simulink model "ASM_Traffic_new"  (R2024a)
settings: Solver=ode1  StartTime=SIM.tstart.v  StopTime=SIM.tend.v  FixedStep=SIM.StepSize.v  RelTol=1e-3
PostLoadFcn:
  | if any(exist('dsrtsu_mdlpostloadfcn', 'file') ~= 0), dsrtsu_mdlpostloadfcn('Execute', bdroot); end
  | try, asm_mdl_postloadfcn(bdroot, 'UpdateModel', 3600); catch, disp(lasterr); end,
InitFcn:
  | , if any(exist('rtifpga_mdlclblib', 'file') ~= 0), rtifpga_mdlclblib('Init', bdroot); end,
  | , if any(exist('dsmpb_private', 'file') ~= 0), dsmpb_private('dsmpb_mdlclblib', 'Init', bdroot); end,
undefined symbols (not defined in the file): _to_, a0b2, ASM_BrakeHydraulics_DemoSystems, ASM_VehicleDynamics_DemoSystems, b98103fe8ad365046cd0, BrakeCircuit, CPT, Crankshaft, DiscIntNeverNeededParam, dsmsi, FinalDriveAssembly, MDL, ModeSignals, Pos_BrakePedal_Maneuver, rad, RefSignals, s_to_rpm, SIM, SoftECU, Suspension, Tire, Transmission
libraries: ASM_Traffic_lib x135, simulink x100, ASM_Utils_lib x77, ASM_VehicleDynamics_lib x70, ASM_Environment_lib x22, dsmpblib x20, dsmsilib x15, MDLD_Utils_lib x10, ASM_BrakeHydraulics_lib x3
(part 45 of 63)

== system ASM_Traffic_new/Drivetrain/Plant/UserInterface/DISP_Plant/ActiveTransmission/Trq_Out_Trm[Nm] ==
  In1 : Inport
  Out1 : Outport  VectorParamsAs1DForOutWhenUnconnected=off
  wires:
  In1/1 -> Out1/1

== system ASM_Traffic_new/Drivetrain/Plant/UserInterface/DISP_Plant/ActiveTransmission/i_Trm[] ==
  In1 : Inport
  Out1 : Outport  VectorParamsAs1DForOutWhenUnconnected=off
  wires:
  In1/1 -> Out1/1

== system ASM_Traffic_new/Drivetrain/Plant/UserInterface/DISP_Plant/ActiveTransmission/i_unsync_Trm[] ==
  In1 : Inport
  Out1 : Outport  VectorParamsAs1DForOutWhenUnconnected=off
  wires:
  In1/1 -> Out1/1

== system ASM_Traffic_new/Drivetrain/Plant/UserInterface/DISP_Plant/ActiveTransmission/omega_In_Trm[rad|s] ==
  In1 : Inport
  Out1 : Outport  VectorParamsAs1DForOutWhenUnconnected=off
  wires:
  In1/1 -> Out1/1

== system ASM_Traffic_new/Drivetrain/Plant/UserInterface/DISP_Plant/ActiveTransmission/omega_Out_Trm[rad|s] ==
  In1 : Inport
  Out1 : Outport  VectorParamsAs1DForOutWhenUnconnected=off
  wires:
  In1/1 -> Out1/1

== system ASM_Traffic_new/Drivetrain/Plant/UserInterface/DISP_Plant/AutomaticTransmission/Trq_Fric_Clutch[Nm] ==
  In1 : Inport
  Out1 : Outport  VectorParamsAs1DForOutWhenUnconnected=off
  wires:
  In1/1 -> Out1/1

== system ASM_Traffic_new/Drivetrain/Plant/UserInterface/DISP_Plant/AutomaticTransmission/Trq_Pump[Nm] ==
  In1 : Inport
  Out1 : Outport  VectorParamsAs1DForOutWhenUnconnected=off
  wires:
  In1/1 -> Out1/1

== system ASM_Traffic_new/Drivetrain/Plant/UserInterface/DISP_Plant/AutomaticTransmission/Trq_TorsionSpring_Clutch[Nm] ==
  In1 : Inport
  Out1 : Outport  VectorParamsAs1DForOutWhenUnconnected=off
  wires:
  In1/1 -> Out1/1

== system ASM_Traffic_new/Drivetrain/Plant/UserInterface/DISP_Plant/AutomaticTransmission/Trq_Turbine[Nm] ==
  In1 : Inport
  Out1 : Outport  VectorParamsAs1DForOutWhenUnconnected=off
  wires:
  In1/1 -> Out1/1

== system ASM_Traffic_new/Drivetrain/Plant/UserInterface/DISP_Plant/AutomaticTransmission/omega_Out_ClutchPlate[rad|s] ==
  In1 : Inport
  Out1 : Outport  VectorParamsAs1DForOutWhenUnconnected=off
  wires:
  In1/1 -> Out1/1

== system ASM_Traffic_new/Drivetrain/Plant/UserInterface/DISP_Plant/EngineSpeed/Trq_Starter[Nm] ==
  In1 : Inport
  Out1 : Outport  VectorParamsAs1DForOutWhenUnconnected=off
  wires:
  In1/1 -> Out1/1

== system ASM_Traffic_new/Drivetrain/Plant/UserInterface/DISP_Plant/EngineSpeed/n_Engine[rpm] ==
  In1 : Inport
  Out1 : Outport  VectorParamsAs1DForOutWhenUnconnected=off
  wires:
  In1/1 -> Out1/1

== system ASM_Traffic_new/Drivetrain/Plant/UserInterface/DISP_Plant/ManualTransmission/Trq_Fric_Clutch[Nm] ==
  In1 : Inport
  Out1 : Outport  VectorParamsAs1DForOutWhenUnconnected=off
  wires:
  In1/1 -> Out1/1

== system ASM_Traffic_new/Drivetrain/Plant/UserInterface/DISP_Plant/ManualTransmission/Trq_TorsionSpring_Clutch[Nm] ==
  In1 : Inport
  Out1 : Outport  VectorParamsAs1DForOutWhenUnconnected=off
  wires:
  In1/1 -> Out1/1

== system ASM_Traffic_new/Drivetrain/Plant/UserInterface/DISP_Plant/ManualTransmission/omega_Out_ClutchPlate[rad|s] ==
  In1 : Inport
  Out1 : Outport  VectorParamsAs1DForOutWhenUnconnected=off
  wires:
  In1/1 -> Out1/1

== system ASM_Traffic_new/Drivetrain/Plant/UserInterface/DISP_Plant/Shafts/Trq_CF_Shaft[Nm] ==
  In1 : Inport
  Out1 : Outport  VectorParamsAs1DForOutWhenUnconnected=off
  wires:
  In1/1 -> Out1/1

== system ASM_Traffic_new/Drivetrain/Plant/UserInterface/DISP_Plant/Shafts/Trq_CR_Shaft[Nm] ==
  In1 : Inport
  Out1 : Outport  VectorParamsAs1DForOutWhenUnconnected=off
  wires:
  In1/1 -> Out1/1

== system ASM_Traffic_new/Drivetrain/Plant/UserInterface/DISP_Plant/Shafts/Trq_FL_Shaft[Nm] ==
  In1 : Inport
  Out1 : Outport  VectorParamsAs1DForOutWhenUnconnected=off
  wires:
  In1/1 -> Out1/1

== system ASM_Traffic_new/Drivetrain/Plant/UserInterface/DISP_Plant/Shafts/Trq_FR_Shaft[Nm] ==
  In1 : Inport
  Out1 : Outport  VectorParamsAs1DForOutWhenUnconnected=off
  wires:
  In1/1 -> Out1/1

== system ASM_Traffic_new/Drivetrain/Plant/UserInterface/DISP_Plant/Shafts/Trq_RL_Shaft[Nm] ==
  In1 : Inport
  Out1 : Outport  VectorParamsAs1DForOutWhenUnconnected=off
  wires:
  In1/1 -> Out1/1

== system ASM_Traffic_new/Drivetrain/Plant/UserInterface/DISP_Plant/Shafts/Trq_RR_Shaft[Nm] ==
  In1 : Inport
  Out1 : Outport  VectorParamsAs1DForOutWhenUnconnected=off
  wires:
  In1/1 -> Out1/1

== system ASM_Traffic_new/Environment/GroundTruth/UserInterface/PAR_Plant/Ego_Vehicle/Indicator_State[] ==
  ASM_Vehicle_TurnLights[] : Inport
  ASM_OSI_Mapping : Subsystem
  Ext_Indicator_State[] : Constant  Value=0
  Multiport Switch : MultiPortSwitch  DataPortOrder=Zero-based contiguous  zeroidx=on  SaturateOnIntegerOverflow=off  InputSameDT=off
  Rounding Function : Rounding  Operator=round
  Saturation : Saturate  UpperLimit=2  LowerLimit=0
  Stim_Indicator_State[] : Constant  Value=0
  Sw_Indicator[0Stim|1Ext|2Mnv] : Constant  Value=2
  Indicator_State[] : Outport  VectorParamsAs1DForOutWhenUnconnected=off
  wires:
  ASM_OSI_Mapping/1(Indicator_State[]) -> Multiport Switch/4  "Mnv_Indicator_State[]"
  Stim_Indicator_State[]/1 -> Multiport Switch/2  "Stim_Indicator_State[]"
  Multiport Switch/1 -> Indicator_State[]/1  "Indicator_State[]"
  Saturation/1 -> Multiport Switch/1
  Rounding Function/1 -> Saturation/1
  Ext_Indicator_State[]/1 -> Multiport Switch/3  "Ext_Indicator_State[]"
  ASM_Vehicle_TurnLights[]/1 -> ASM_OSI_Mapping/1(ASM_Vehicle_TurnLights[])
  Sw_Indicator[0Stim|1Ext|2Mnv]/1 -> Rounding Function/1  "Sw_Indicator[0Stim|1Ext|2Mnv]"

== system ASM_Traffic_new/Environment/GroundTruth/UserInterface/PAR_Plant/Fellow_Vehicles/Demux_Fellow_Lightstates ==
  Fellow_Lightstates[] : Inport
  Add{,1..8} (9 alike) : Sum
  Constant : Constant
  Constant1 : Constant  Value=2
  Constant2 : Constant  Value=3
  Constant3 : Constant  Value=4
  Constant4 : Constant  Value=5
  Constant5 : Constant  Value=8
  Constant6 : Constant  Value=9
  Constant7 : Constant  Value=6
  Constant8 : Constant  Value=7
  Main_Idx_30Fellows : Constant  Value=[1,11,21,31,41,51,61,71,81,91,101,111,121,131,141,151,161,171,181,191,201,211,221,231,241,251,261,271,281,291]
  Selector_Brake_State[] : Selector  InputPortWidth=MDL.Traffic.MaxNumFellows.v*10  IndexOptions=Index vector (port)  Indices=[1 3]  OutputSizes=1
  Selector_Emergency_Veh_Illu[] : Selector  InputPortWidth=MDL.Traffic.MaxNumFellows.v*10  IndexOptions=Index vector (port)  Indices=[1 3]  OutputSizes=1
  Selector_Front_Fog_Light[] : Selector  InputPortWidth=MDL.Traffic.MaxNumFellows.v*10  IndexOptions=Index vector (port)  Indices=[1 3]  OutputSizes=1
  Selector_Head_Light[] : Selector  InputPortWidth=MDL.Traffic.MaxNumFellows.v*10  IndexOptions=Index vector (port)  Indices=[1 3]  OutputSizes=1
  Selector_High_Beam : Selector  InputPortWidth=MDL.Traffic.MaxNumFellows.v*10  IndexOptions=Index vector (port)  Indices=[1 3]  OutputSizes=1
  Selector_Indicator_State[] : Selector  InputPortWidth=MDL.Traffic.MaxNumFellows.v*10  IndexOptions=Index vector (port)  Indices=[1 3]  OutputSizes=1
  Selector_License_Plate_Illumination[] : Selector  InputPortWidth=MDL.Traffic.MaxNumFellows.v*10  IndexOptions=Index vector (port)  Indices=[1 3]  OutputSizes=1
  Selector_Rear_Fog_Light[] : Selector  InputPortWidth=MDL.Traffic.MaxNumFellows.v*10  IndexOptions=Index vector (port)  Indices=[1 3]  OutputSizes=1
  Selector_Reversing_Light[] : Selector  InputPortWidth=MDL.Traffic.MaxNumFellows.v*10  IndexOptions=Index vector (port)  Indices=[1 3]  OutputSizes=1
  Selector_Service_Veh_Illu[] : Selector  InputPortWidth=MDL.Traffic.MaxNumFellows.v*10  IndexOptions=Index vector (port)  Indices=[1 3]  OutputSizes=1
  High_Beam_Fellows[] : Outport  VectorParamsAs1DForOutWhenUnconnected=off
  Reversing_Light_Fellows[] : Outport  Port=2  VectorParamsAs1DForOutWhenUnconnected=off
  Front_Fog_Light_Fellows[] : Outport  Port=3  VectorParamsAs1DForOutWhenUnconnected=off
  Head_Light_Fellows[] : Outport  Port=4  VectorParamsAs1DForOutWhenUnconnected=off
  License_Plate_Illumination_Fellows[] : Outport  Port=5  VectorParamsAs1DForOutWhenUnconnected=off
  Rear_Fog_Light_Fellows[] : Outport  Port=6  VectorParamsAs1DForOutWhenUnconnected=off
  Emergency_Veh_Illu_Fellows[] : Outport  Port=7  VectorParamsAs1DForOutWhenUnconnected=off
  Service_Veh_Illu_Fellows[] : Outport  Port=8  VectorParamsAs1DForOutWhenUnconnected=off
  Indicator_State_Fellows[] : Outport  Port=9  VectorParamsAs1DForOutWhenUnconnected=off
  Brake_Fellows[] : Outport  Port=10  VectorParamsAs1DForOutWhenUnconnected=off
  wires:
  Fellow_Lightstates[]/1 -> Selector_Service_Veh_Illu[]/1, Selector_Brake_State[]/1, Selector_Indicator_State[]/1, Selector_Emergency_Veh_Illu[]/1, Selector_Rear_Fog_Light[]/1, Selector_License_Plate_Illumination[]/1, Selector_Head_Light[]/1, Selector_Front_Fog_Light[]/1, Selector_Reversing_Light[]/1, Selector_High_Beam/1
  Main_Idx_30Fellows/1 -> Add7/1, Add8/1, Add6/1, Add5/1, Add4/1, Add3/1, Add2/1, Add1/1, Add/1, Selector_High_Beam/2
  Selector_High_Beam/1 -> High_Beam_Fellows[]/1
  Add/1 -> Selector_Reversing_Light[]/2
  Constant/1 -> Add/2
  Selector_Reversing_Light[]/1 -> Reversing_Light_Fellows[]/1
  Selector_Front_Fog_Light[]/1 -> Front_Fog_Light_Fellows[]/1
  Add1/1 -> Selector_Front_Fog_Light[]/2
  Constant1/1 -> Add1/2
  Selector_Head_Light[]/1 -> Head_Light_Fellows[]/1
  Add2/1 -> Selector_Head_Light[]/2
  Constant2/1 -> Add2/2
  Selector_License_Plate_Illumination[]/1 -> License_Plate_Illumination_Fellows[]/1
  Add3/1 -> Selector_License_Plate_Illumination[]/2
  Constant3/1 -> Add3/2
  Selector_Rear_Fog_Light[]/1 -> Rear_Fog_Light_Fellows[]/1
  Add4/1 -> Selector_Rear_Fog_Light[]/2
  Constant4/1 -> Add4/2
  Selector_Indicator_State[]/1 -> Indicator_State_Fellows[]/1
  Add5/1 -> Selector_Indicator_State[]/2
  Constant5/1 -> Add5/2
  Selector_Brake_State[]/1 -> Brake_Fellows[]/1
  Add6/1 -> Selector_Brake_State[]/2
  Constant6/1 -> Add6/2
  Add7/1 -> Selector_Emergency_Veh_Illu[]/2
  Constant7/1 -> Add7/2
  Add8/1 -> Selector_Service_Veh_Illu[]/2
  Constant8/1 -> Add8/2
  Selector_Emergency_Veh_Illu[]/1 -> Emergency_Veh_Illu_Fellows[]/1
  Selector_Service_Veh_Illu[]/1 -> Service_Veh_Illu_Fellows[]/1

== system ASM_Traffic_new/Environment/GroundTruth/UserInterface/PAR_Plant/Fellow_Vehicles/Lightstates_Fellow1 ==
  Fellow_Indicator_State[] : Inport
  Brake[] : Constant  Tag=AD:ASM_Sw_SpeedLimit_Source[1Manual|2RoadScenery]  Value=2
  Emergency_Vehicle_Illumination[] : Constant  Tag=AD:ASM_Sw_SpeedLimit_Source[1Manual|2RoadScenery]  Value=2
  Front_Fog_Light[] : Constant  Tag=AD:ASM_Sw_SpeedLimit_Source[1Manual|2RoadScenery]  Value=2
  Head_Light[] : Constant  Tag=AD:ASM_Sw_SpeedLimit_Source[1Manual|2RoadScenery]  Value=2
  High_Beam[] : Constant  Tag=AD:ASM_Sw_SpeedLimit_Source[1Manual|2RoadScenery]  Value=2
  Indicator_State[] : Subsystem
  License_Plate_Illumination_Rear[] : Constant  Tag=AD:ASM_Sw_SpeedLimit_Source[1Manual|2RoadScenery]  Value=2
  Mux : Mux  Inputs=10
  Rear_Fog_Light[] : Constant  Tag=AD:ASM_Sw_SpeedLimit_Source[1Manual|2RoadScenery]  Value=2
  Reversing_Light[] : Constant  Tag=AD:ASM_Sw_SpeedLimit_Source[1Manual|2RoadScenery]  Value=2
  Service_Vehicle_Illumination[] : Constant  Tag=AD:ASM_Sw_SpeedLimit_Source[1Manual|2RoadScenery]  Value=2
  Lightstates[] : Outport  VectorParamsAs1DForOutWhenUnconnected=off
  wires:
  Fellow_Indicator_State[]/1 -> Indicator_State[]/1(Fellow_TurnLights[])
  Mux/1 -> Lightstates[]/1  "LightStates[]"
  Indicator_State[]/1(Indicator_State[]) -> Mux/9
  Reversing_Light[]/1 -> Mux/2
  High_Beam[]/1 -> Mux/1
  Head_Light[]/1 -> Mux/4
  Brake[]/1 -> Mux/10
  Rear_Fog_Light[]/1 -> Mux/6
  Front_Fog_Light[]/1 -> Mux/3
  License_Plate_Illumination_Rear[]/1 -> Mux/5
  Emergency_Vehicle_Illumination[]/1 -> Mux/7
  Service_Vehicle_Illumination[]/1 -> Mux/8

== system ASM_Traffic_new/Environment/GroundTruth/UserInterface/PAR_Plant/Fellow_Vehicles/Lightstates_Fellow10 ==
  Fellow_Indicator_State[] : Inport
  Brake[] : Constant  Tag=AD:ASM_Sw_SpeedLimit_Source[1Manual|2RoadScenery]  Value=2
  Emergency_Vehicle_Illumination[] : Constant  Tag=AD:ASM_Sw_SpeedLimit_Source[1Manual|2RoadScenery]  Value=2
  Front_Fog_Light[] : Constant  Tag=AD:ASM_Sw_SpeedLimit_Source[1Manual|2RoadScenery]  Value=2
  Head_Light[] : Constant  Tag=AD:ASM_Sw_SpeedLimit_Source[1Manual|2RoadScenery]  Value=2
  High_Beam[] : Constant  Tag=AD:ASM_Sw_SpeedLimit_Source[1Manual|2RoadScenery]  Value=2
  Indicator_State[] : Subsystem
  License_Plate_Illumination_Rear[] : Constant  Tag=AD:ASM_Sw_SpeedLimit_Source[1Manual|2RoadScenery]  Value=2
  Mux : Mux  Inputs=10
  Rear_Fog_Light[] : Constant  Tag=AD:ASM_Sw_SpeedLimit_Source[1Manual|2RoadScenery]  Value=2
  Reversing_Light[] : Constant  Tag=AD:ASM_Sw_SpeedLimit_Source[1Manual|2RoadScenery]  Value=2
  Service_Vehicle_Illumination[] : Constant  Tag=AD:ASM_Sw_SpeedLimit_Source[1Manual|2RoadScenery]  Value=2
  Lightstates[] : Outport  VectorParamsAs1DForOutWhenUnconnected=off
  wires:
  Service_Vehicle_Illumination[]/1 -> Mux/8
  Emergency_Vehicle_Illumination[]/1 -> Mux/7
  License_Plate_Illumination_Rear[]/1 -> Mux/5
  Front_Fog_Light[]/1 -> Mux/3
  Rear_Fog_Light[]/1 -> Mux/6
  Brake[]/1 -> Mux/10
  Head_Light[]/1 -> Mux/4
  High_Beam[]/1 -> Mux/1
  Reversing_Light[]/1 -> Mux/2
  Indicator_State[]/1(Indicator_State[]) -> Mux/9
  Mux/1 -> Lightstates[]/1  "LightStates[]"
  Fellow_Indicator_State[]/1 -> Indicator_State[]/1(Fellow_TurnLights[])

== system ASM_Traffic_new/Environment/GroundTruth/UserInterface/PAR_Plant/Fellow_Vehicles/Lightstates_Fellow11 ==
  Fellow_Indicator_State[] : Inport
  Brake[] : Constant  Tag=AD:ASM_Sw_SpeedLimit_Source[1Manual|2RoadScenery]  Value=2
  Emergency_Vehicle_Illumination[] : Constant  Tag=AD:ASM_Sw_SpeedLimit_Source[1Manual|2RoadScenery]  Value=2
  Front_Fog_Light[] : Constant  Tag=AD:ASM_Sw_SpeedLimit_Source[1Manual|2RoadScenery]  Value=2
  Head_Light[] : Constant  Tag=AD:ASM_Sw_SpeedLimit_Source[1Manual|2RoadScenery]  Value=2
  High_Beam[] : Constant  Tag=AD:ASM_Sw_SpeedLimit_Source[1Manual|2RoadScenery]  Value=2
  Indicator_State[] : Subsystem
  License_Plate_Illumination_Rear[] : Constant  Tag=AD:ASM_Sw_SpeedLimit_Source[1Manual|2RoadScenery]  Value=2
  Mux : Mux  Inputs=10
  Rear_Fog_Light[] : Constant  Tag=AD:ASM_Sw_SpeedLimit_Source[1Manual|2RoadScenery]  Value=2
  Reversing_Light[] : Constant  Tag=AD:ASM_Sw_SpeedLimit_Source[1Manual|2RoadScenery]  Value=2
  Service_Vehicle_Illumination[] : Constant  Tag=AD:ASM_Sw_SpeedLimit_Source[1Manual|2RoadScenery]  Value=2
  Lightstates[] : Outport  VectorParamsAs1DForOutWhenUnconnected=off
  wires:
  Fellow_Indicator_State[]/1 -> Indicator_State[]/1(Fellow_TurnLights[])
  Mux/1 -> Lightstates[]/1  "LightStates[]"
  Indicator_State[]/1(Indicator_State[]) -> Mux/9
  Reversing_Light[]/1 -> Mux/2
  High_Beam[]/1 -> Mux/1
  Head_Light[]/1 -> Mux/4
  Brake[]/1 -> Mux/10
  Rear_Fog_Light[]/1 -> Mux/6
  Front_Fog_Light[]/1 -> Mux/3
  License_Plate_Illumination_Rear[]/1 -> Mux/5
  Emergency_Vehicle_Illumination[]/1 -> Mux/7
  Service_Vehicle_Illumination[]/1 -> Mux/8

== system ASM_Traffic_new/Environment/GroundTruth/UserInterface/PAR_Plant/Fellow_Vehicles/Lightstates_Fellow12 ==
  Fellow_Indicator_State[] : Inport
  Brake[] : Constant  Tag=AD:ASM_Sw_SpeedLimit_Source[1Manual|2RoadScenery]  Value=2
  Emergency_Vehicle_Illumination[] : Constant  Tag=AD:ASM_Sw_SpeedLimit_Source[1Manual|2RoadScenery]  Value=2
  Front_Fog_Light[] : Constant  Tag=AD:ASM_Sw_SpeedLimit_Source[1Manual|2RoadScenery]  Value=2
  Head_Light[] : Constant  Tag=AD:ASM_Sw_SpeedLimit_Source[1Manual|2RoadScenery]  Value=2
  High_Beam[] : Constant  Tag=AD:ASM_Sw_SpeedLimit_Source[1Manual|2RoadScenery]  Value=2
  Indicator_State[] : Subsystem
  License_Plate_Illumination_Rear[] : Constant  Tag=AD:ASM_Sw_SpeedLimit_Source[1Manual|2RoadScenery]  Value=2
  Mux : Mux  Inputs=10
  Rear_Fog_Light[] : Constant  Tag=AD:ASM_Sw_SpeedLimit_Source[1Manual|2RoadScenery]  Value=2
  Reversing_Light[] : Constant  Tag=AD:ASM_Sw_SpeedLimit_Source[1Manual|2RoadScenery]  Value=2
  Service_Vehicle_Illumination[] : Constant  Tag=AD:ASM_Sw_SpeedLimit_Source[1Manual|2RoadScenery]  Value=2
  Lightstates[] : Outport  VectorParamsAs1DForOutWhenUnconnected=off
  wires:
  Service_Vehicle_Illumination[]/1 -> Mux/8
  Emergency_Vehicle_Illumination[]/1 -> Mux/7
  License_Plate_Illumination_Rear[]/1 -> Mux/5
  Front_Fog_Light[]/1 -> Mux/3
  Rear_Fog_Light[]/1 -> Mux/6
  Brake[]/1 -> Mux/10
  Head_Light[]/1 -> Mux/4
  High_Beam[]/1 -> Mux/1
  Reversing_Light[]/1 -> Mux/2
  Indicator_State[]/1(Indicator_State[]) -> Mux/9
  Mux/1 -> Lightstates[]/1  "LightStates[]"
  Fellow_Indicator_State[]/1 -> Indicator_State[]/1(Fellow_TurnLights[])

== system ASM_Traffic_new/Environment/GroundTruth/UserInterface/PAR_Plant/Fellow_Vehicles/Lightstates_Fellow13 ==
  Fellow_Indicator_State[] : Inport
  Brake[] : Constant  Tag=AD:ASM_Sw_SpeedLimit_Source[1Manual|2RoadScenery]  Value=2
  Emergency_Vehicle_Illumination[] : Constant  Tag=AD:ASM_Sw_SpeedLimit_Source[1Manual|2RoadScenery]  Value=2
  Front_Fog_Light[] : Constant  Tag=AD:ASM_Sw_SpeedLimit_Source[1Manual|2RoadScenery]  Value=2
  Head_Light[] : Constant  Tag=AD:ASM_Sw_SpeedLimit_Source[1Manual|2RoadScenery]  Value=2
  High_Beam[] : Constant  Tag=AD:ASM_Sw_SpeedLimit_Source[1Manual|2RoadScenery]  Value=2
  Indicator_State[] : Subsystem
  License_Plate_Illumination_Rear[] : Constant  Tag=AD:ASM_Sw_SpeedLimit_Source[1Manual|2RoadScenery]  Value=2
  Mux : Mux  Inputs=10
  Rear_Fog_Light[] : Constant  Tag=AD:ASM_Sw_SpeedLimit_Source[1Manual|2RoadScenery]  Value=2
  Reversing_Light[] : Constant  Tag=AD:ASM_Sw_SpeedLimit_Source[1Manual|2RoadScenery]  Value=2
  Service_Vehicle_Illumination[] : Constant  Tag=AD:ASM_Sw_SpeedLimit_Source[1Manual|2RoadScenery]  Value=2
  Lightstates[] : Outport  VectorParamsAs1DForOutWhenUnconnected=off
  wires:
  Fellow_Indicator_State[]/1 -> Indicator_State[]/1(Fellow_TurnLights[])
  Mux/1 -> Lightstates[]/1  "LightStates[]"
  Indicator_State[]/1(Indicator_State[]) -> Mux/9
  Reversing_Light[]/1 -> Mux/2
  High_Beam[]/1 -> Mux/1
  Head_Light[]/1 -> Mux/4
  Brake[]/1 -> Mux/10
  Rear_Fog_Light[]/1 -> Mux/6
  Front_Fog_Light[]/1 -> Mux/3
  License_Plate_Illumination_Rear[]/1 -> Mux/5
  Emergency_Vehicle_Illumination[]/1 -> Mux/7
  Service_Vehicle_Illumination[]/1 -> Mux/8

== system ASM_Traffic_new/Environment/GroundTruth/UserInterface/PAR_Plant/Fellow_Vehicles/Lightstates_Fellow14 ==
  Fellow_Indicator_State[] : Inport
  Brake[] : Constant  Tag=AD:ASM_Sw_SpeedLimit_Source[1Manual|2RoadScenery]  Value=2
  Emergency_Vehicle_Illumination[] : Constant  Tag=AD:ASM_Sw_SpeedLimit_Source[1Manual|2RoadScenery]  Value=2
  Front_Fog_Light[] : Constant  Tag=AD:ASM_Sw_SpeedLimit_Source[1Manual|2RoadScenery]  Value=2
  Head_Light[] : Constant  Tag=AD:ASM_Sw_SpeedLimit_Source[1Manual|2RoadScenery]  Value=2
  High_Beam[] : Constant  Tag=AD:ASM_Sw_SpeedLimit_Source[1Manual|2RoadScenery]  Value=2
  Indicator_State[] : Subsystem
  License_Plate_Illumination_Rear[] : Constant  Tag=AD:ASM_Sw_SpeedLimit_Source[1Manual|2RoadScenery]  Value=2
  Mux : Mux  Inputs=10
  Rear_Fog_Light[] : Constant  Tag=AD:ASM_Sw_SpeedLimit_Source[1Manual|2RoadScenery]  Value=2
  Reversing_Light[] : Constant  Tag=AD:ASM_Sw_SpeedLimit_Source[1Manual|2RoadScenery]  Value=2
  Service_Vehicle_Illumination[] : Constant  Tag=AD:ASM_Sw_SpeedLimit_Source[1Manual|2RoadScenery]  Value=2
  Lightstates[] : Outport  VectorParamsAs1DForOutWhenUnconnected=off
  wires:
  Service_Vehicle_Illumination[]/1 -> Mux/8
  Emergency_Vehicle_Illumination[]/1 -> Mux/7
  License_Plate_Illumination_Rear[]/1 -> Mux/5
  Front_Fog_Light[]/1 -> Mux/3
  Rear_Fog_Light[]/1 -> Mux/6
  Brake[]/1 -> Mux/10
  Head_Light[]/1 -> Mux/4
  High_Beam[]/1 -> Mux/1
  Reversing_Light[]/1 -> Mux/2
  Indicator_State[]/1(Indicator_State[]) -> Mux/9
  Mux/1 -> Lightstates[]/1  "LightStates[]"
  Fellow_Indicator_State[]/1 -> Indicator_State[]/1(Fellow_TurnLights[])

== system ASM_Traffic_new/Environment/GroundTruth/UserInterface/PAR_Plant/Fellow_Vehicles/Lightstates_Fellow15 ==
  Fellow_Indicator_State[] : Inport
  Brake[] : Constant  Tag=AD:ASM_Sw_SpeedLimit_Source[1Manual|2RoadScenery]  Value=2
  Emergency_Vehicle_Illumination[] : Constant  Tag=AD:ASM_Sw_SpeedLimit_Source[1Manual|2RoadScenery]  Value=2
  Front_Fog_Light[] : Constant  Tag=AD:ASM_Sw_SpeedLimit_Source[1Manual|2RoadScenery]  Value=2
  Head_Light[] : Constant  Tag=AD:ASM_Sw_SpeedLimit_Source[1Manual|2RoadScenery]  Value=2
  High_Beam[] : Constant  Tag=AD:ASM_Sw_SpeedLimit_Source[1Manual|2RoadScenery]  Value=2
  Indicator_State[] : Subsystem
  License_Plate_Illumination_Rear[] : Constant  Tag=AD:ASM_Sw_SpeedLimit_Source[1Manual|2RoadScenery]  Value=2
  Mux : Mux  Inputs=10
  Rear_Fog_Light[] : Constant  Tag=AD:ASM_Sw_SpeedLimit_Source[1Manual|2RoadScenery]  Value=2
  Reversing_Light[] : Constant  Tag=AD:ASM_Sw_SpeedLimit_Source[1Manual|2RoadScenery]  Value=2
  Service_Vehicle_Illumination[] : Constant  Tag=AD:ASM_Sw_SpeedLimit_Source[1Manual|2RoadScenery]  Value=2
  Lightstates[] : Outport  VectorParamsAs1DForOutWhenUnconnected=off
  wires:
  Fellow_Indicator_State[]/1 -> Indicator_State[]/1(Fellow_TurnLights[])
  Mux/1 -> Lightstates[]/1  "LightStates[]"
  Indicator_State[]/1(Indicator_State[]) -> Mux/9
  Reversing_Light[]/1 -> Mux/2
  High_Beam[]/1 -> Mux/1
  Head_Light[]/1 -> Mux/4
  Brake[]/1 -> Mux/10
  Rear_Fog_Light[]/1 -> Mux/6
  Front_Fog_Light[]/1 -> Mux/3
  License_Plate_Illumination_Rear[]/1 -> Mux/5
  Emergency_Vehicle_Illumination[]/1 -> Mux/7
  Service_Vehicle_Illumination[]/1 -> Mux/8

== system ASM_Traffic_new/Environment/GroundTruth/UserInterface/PAR_Plant/Fellow_Vehicles/Lightstates_Fellow16 ==
  Fellow_Indicator_State[] : Inport
  Brake[] : Constant  Tag=AD:ASM_Sw_SpeedLimit_Source[1Manual|2RoadScenery]  Value=2
  Emergency_Vehicle_Illumination[] : Constant  Tag=AD:ASM_Sw_SpeedLimit_Source[1Manual|2RoadScenery]  Value=2
  Front_Fog_Light[] : Constant  Tag=AD:ASM_Sw_SpeedLimit_Source[1Manual|2RoadScenery]  Value=2
  Head_Light[] : Constant  Tag=AD:ASM_Sw_SpeedLimit_Source[1Manual|2RoadScenery]  Value=2
  High_Beam[] : Constant  Tag=AD:ASM_Sw_SpeedLimit_Source[1Manual|2RoadScenery]  Value=2
  Indicator_State[] : Subsystem
  License_Plate_Illumination_Rear[] : Constant  Tag=AD:ASM_Sw_SpeedLimit_Source[1Manual|2RoadScenery]  Value=2
  Mux : Mux  Inputs=10
  Rear_Fog_Light[] : Constant  Tag=AD:ASM_Sw_SpeedLimit_Source[1Manual|2RoadScenery]  Value=2
  Reversing_Light[] : Constant  Tag=AD:ASM_Sw_SpeedLimit_Source[1Manual|2RoadScenery]  Value=2
  Service_Vehicle_Illumination[] : Constant  Tag=AD:ASM_Sw_SpeedLimit_Source[1Manual|2RoadScenery]  Value=2
  Lightstates[] : Outport  VectorParamsAs1DForOutWhenUnconnected=off
  wires:
  Service_Vehicle_Illumination[]/1 -> Mux/8
  Emergency_Vehicle_Illumination[]/1 -> Mux/7
  License_Plate_Illumination_Rear[]/1 -> Mux/5
  Front_Fog_Light[]/1 -> Mux/3
  Rear_Fog_Light[]/1 -> Mux/6
  Brake[]/1 -> Mux/10
  Head_Light[]/1 -> Mux/4
  High_Beam[]/1 -> Mux/1
  Reversing_Light[]/1 -> Mux/2
  Indicator_State[]/1(Indicator_State[]) -> Mux/9
  Mux/1 -> Lightstates[]/1  "LightStates[]"
  Fellow_Indicator_State[]/1 -> Indicator_State[]/1(Fellow_TurnLights[])

== system ASM_Traffic_new/Environment/GroundTruth/UserInterface/PAR_Plant/Fellow_Vehicles/Lightstates_Fellow17 ==
  Fellow_Indicator_State[] : Inport
  Brake[] : Constant  Tag=AD:ASM_Sw_SpeedLimit_Source[1Manual|2RoadScenery]  Value=2
  Emergency_Vehicle_Illumination[] : Constant  Tag=AD:ASM_Sw_SpeedLimit_Source[1Manual|2RoadScenery]  Value=2
  Front_Fog_Light[] : Constant  Tag=AD:ASM_Sw_SpeedLimit_Source[1Manual|2RoadScenery]  Value=2
  Head_Light[] : Constant  Tag=AD:ASM_Sw_SpeedLimit_Source[1Manual|2RoadScenery]  Value=2
  High_Beam[] : Constant  Tag=AD:ASM_Sw_SpeedLimit_Source[1Manual|2RoadScenery]  Value=2
  Indicator_State[] : Subsystem
  License_Plate_Illumination_Rear[] : Constant  Tag=AD:ASM_Sw_SpeedLimit_Source[1Manual|2RoadScenery]  Value=2
  Mux : Mux  Inputs=10
  Rear_Fog_Light[] : Constant  Tag=AD:ASM_Sw_SpeedLimit_Source[1Manual|2RoadScenery]  Value=2
  Reversing_Light[] : Constant  Tag=AD:ASM_Sw_SpeedLimit_Source[1Manual|2RoadScenery]  Value=2
  Service_Vehicle_Illumination[] : Constant  Tag=AD:ASM_Sw_SpeedLimit_Source[1Manual|2RoadScenery]  Value=2
  Lightstates[] : Outport  VectorParamsAs1DForOutWhenUnconnected=off
  wires:
  Fellow_Indicator_State[]/1 -> Indicator_State[]/1(Fellow_TurnLights[])
  Mux/1 -> Lightstates[]/1  "LightStates[]"
  Indicator_State[]/1(Indicator_State[]) -> Mux/9
  Reversing_Light[]/1 -> Mux/2
  High_Beam[]/1 -> Mux/1
  Head_Light[]/1 -> Mux/4
  Brake[]/1 -> Mux/10
  Rear_Fog_Light[]/1 -> Mux/6
  Front_Fog_Light[]/1 -> Mux/3
  License_Plate_Illumination_Rear[]/1 -> Mux/5
  Emergency_Vehicle_Illumination[]/1 -> Mux/7
  Service_Vehicle_Illumination[]/1 -> Mux/8

== system ASM_Traffic_new/Environment/GroundTruth/UserInterface/PAR_Plant/Fellow_Vehicles/Lightstates_Fellow18 ==
  Fellow_Indicator_State[] : Inport
  Brake[] : Constant  Tag=AD:ASM_Sw_SpeedLimit_Source[1Manual|2RoadScenery]  Value=2
  Emergency_Vehicle_Illumination[] : Constant  Tag=AD:ASM_Sw_SpeedLimit_Source[1Manual|2RoadScenery]  Value=2
  Front_Fog_Light[] : Constant  Tag=AD:ASM_Sw_SpeedLimit_Source[1Manual|2RoadScenery]  Value=2
  Head_Light[] : Constant  Tag=AD:ASM_Sw_SpeedLimit_Source[1Manual|2RoadScenery]  Value=2
  High_Beam[] : Constant  Tag=AD:ASM_Sw_SpeedLimit_Source[1Manual|2RoadScenery]  Value=2
  Indicator_State[] : Subsystem
  License_Plate_Illumination_Rear[] : Constant  Tag=AD:ASM_Sw_SpeedLimit_Source[1Manual|2RoadScenery]  Value=2
  Mux : Mux  Inputs=10
  Rear_Fog_Light[] : Constant  Tag=AD:ASM_Sw_SpeedLimit_Source[1Manual|2RoadScenery]  Value=2
  Reversing_Light[] : Constant  Tag=AD:ASM_Sw_SpeedLimit_Source[1Manual|2RoadScenery]  Value=2
  Service_Vehicle_Illumination[] : Constant  Tag=AD:ASM_Sw_SpeedLimit_Source[1Manual|2RoadScenery]  Value=2
  Lightstates[] : Outport  VectorParamsAs1DForOutWhenUnconnected=off
  wires:
  Service_Vehicle_Illumination[]/1 -> Mux/8
  Emergency_Vehicle_Illumination[]/1 -> Mux/7
  License_Plate_Illumination_Rear[]/1 -> Mux/5
  Front_Fog_Light[]/1 -> Mux/3
  Rear_Fog_Light[]/1 -> Mux/6
  Brake[]/1 -> Mux/10
  Head_Light[]/1 -> Mux/4
  High_Beam[]/1 -> Mux/1
  Reversing_Light[]/1 -> Mux/2
  Indicator_State[]/1(Indicator_State[]) -> Mux/9
  Mux/1 -> Lightstates[]/1  "LightStates[]"
  Fellow_Indicator_State[]/1 -> Indicator_State[]/1(Fellow_TurnLights[])

== system ASM_Traffic_new/Environment/GroundTruth/UserInterface/PAR_Plant/Fellow_Vehicles/Lightstates_Fellow19 ==
  Fellow_Indicator_State[] : Inport
  Brake[] : Constant  Tag=AD:ASM_Sw_SpeedLimit_Source[1Manual|2RoadScenery]  Value=2
  Emergency_Vehicle_Illumination[] : Constant  Tag=AD:ASM_Sw_SpeedLimit_Source[1Manual|2RoadScenery]  Value=2
  Front_Fog_Light[] : Constant  Tag=AD:ASM_Sw_SpeedLimit_Source[1Manual|2RoadScenery]  Value=2
  Head_Light[] : Constant  Tag=AD:ASM_Sw_SpeedLimit_Source[1Manual|2RoadScenery]  Value=2
  High_Beam[] : Constant  Tag=AD:ASM_Sw_SpeedLimit_Source[1Manual|2RoadScenery]  Value=2
  Indicator_State[] : Subsystem
  License_Plate_Illumination_Rear[] : Constant  Tag=AD:ASM_Sw_SpeedLimit_Source[1Manual|2RoadScenery]  Value=2
  Mux : Mux  Inputs=10
  Rear_Fog_Light[] : Constant  Tag=AD:ASM_Sw_SpeedLimit_Source[1Manual|2RoadScenery]  Value=2
  Reversing_Light[] : Constant  Tag=AD:ASM_Sw_SpeedLimit_Source[1Manual|2RoadScenery]  Value=2
  Service_Vehicle_Illumination[] : Constant  Tag=AD:ASM_Sw_SpeedLimit_Source[1Manual|2RoadScenery]  Value=2
  Lightstates[] : Outport  VectorParamsAs1DForOutWhenUnconnected=off
  wires:
  Fellow_Indicator_State[]/1 -> Indicator_State[]/1(Fellow_TurnLights[])
  Mux/1 -> Lightstates[]/1  "LightStates[]"
  Indicator_State[]/1(Indicator_State[]) -> Mux/9
  Reversing_Light[]/1 -> Mux/2
  High_Beam[]/1 -> Mux/1
  Head_Light[]/1 -> Mux/4
  Brake[]/1 -> Mux/10
  Rear_Fog_Light[]/1 -> Mux/6
  Front_Fog_Light[]/1 -> Mux/3
  License_Plate_Illumination_Rear[]/1 -> Mux/5
  Emergency_Vehicle_Illumination[]/1 -> Mux/7
  Service_Vehicle_Illumination[]/1 -> Mux/8

== system ASM_Traffic_new/Environment/GroundTruth/UserInterface/PAR_Plant/Fellow_Vehicles/Lightstates_Fellow2 ==
  Fellow_Indicator_State[] : Inport
  Brake[] : Constant  Tag=AD:ASM_Sw_SpeedLimit_Source[1Manual|2RoadScenery]  Value=2
  Emergency_Vehicle_Illumination[] : Constant  Tag=AD:ASM_Sw_SpeedLimit_Source[1Manual|2RoadScenery]  Value=2
  Front_Fog_Light[] : Constant  Tag=AD:ASM_Sw_SpeedLimit_Source[1Manual|2RoadScenery]  Value=2
  Head_Light[] : Constant  Tag=AD:ASM_Sw_SpeedLimit_Source[1Manual|2RoadScenery]  Value=2
  High_Beam[] : Constant  Tag=AD:ASM_Sw_SpeedLimit_Source[1Manual|2RoadScenery]  Value=2
  Indicator_State[] : Subsystem
  License_Plate_Illumination_Rear[] : Constant  Tag=AD:ASM_Sw_SpeedLimit_Source[1Manual|2RoadScenery]  Value=2
  Mux : Mux  Inputs=10
  Rear_Fog_Light[] : Constant  Tag=AD:ASM_Sw_SpeedLimit_Source[1Manual|2RoadScenery]  Value=2
  Reversing_Light[] : Constant  Tag=AD:ASM_Sw_SpeedLimit_Source[1Manual|2RoadScenery]  Value=2
  Service_Vehicle_Illumination[] : Constant  Tag=AD:ASM_Sw_SpeedLimit_Source[1Manual|2RoadScenery]  Value=2
  Lightstates[] : Outport  VectorParamsAs1DForOutWhenUnconnected=off
  wires:
  Service_Vehicle_Illumination[]/1 -> Mux/8
  Emergency_Vehicle_Illumination[]/1 -> Mux/7
  License_Plate_Illumination_Rear[]/1 -> Mux/5
  Front_Fog_Light[]/1 -> Mux/3
  Rear_Fog_Light[]/1 -> Mux/6
  Brake[]/1 -> Mux/10
  Head_Light[]/1 -> Mux/4
  High_Beam[]/1 -> Mux/1
  Reversing_Light[]/1 -> Mux/2
  Indicator_State[]/1(Indicator_State[]) -> Mux/9
  Mux/1 -> Lightstates[]/1  "LightStates[]"
  Fellow_Indicator_State[]/1 -> Indicator_State[]/1(Fellow_TurnLights[])

== system ASM_Traffic_new/Environment/GroundTruth/UserInterface/PAR_Plant/Fellow_Vehicles/Lightstates_Fellow20 ==
  Fellow_Indicator_State[] : Inport
  Brake[] : Constant  Tag=AD:ASM_Sw_SpeedLimit_Source[1Manual|2RoadScenery]  Value=2
  Emergency_Vehicle_Illumination[] : Constant  Tag=AD:ASM_Sw_SpeedLimit_Source[1Manual|2RoadScenery]  Value=2
  Front_Fog_Light[] : Constant  Tag=AD:ASM_Sw_SpeedLimit_Source[1Manual|2RoadScenery]  Value=2
  Head_Light[] : Constant  Tag=AD:ASM_Sw_SpeedLimit_Source[1Manual|2RoadScenery]  Value=2
  High_Beam[] : Constant  Tag=AD:ASM_Sw_SpeedLimit_Source[1Manual|2RoadScenery]  Value=2
  Indicator_State[] : Subsystem
  License_Plate_Illumination_Rear[] : Constant  Tag=AD:ASM_Sw_SpeedLimit_Source[1Manual|2RoadScenery]  Value=2
  Mux : Mux  Inputs=10
  Rear_Fog_Light[] : Constant  Tag=AD:ASM_Sw_SpeedLimit_Source[1Manual|2RoadScenery]  Value=2
  Reversing_Light[] : Constant  Tag=AD:ASM_Sw_SpeedLimit_Source[1Manual|2RoadScenery]  Value=2
  Service_Vehicle_Illumination[] : Constant  Tag=AD:ASM_Sw_SpeedLimit_Source[1Manual|2RoadScenery]  Value=2
  Lightstates[] : Outport  VectorParamsAs1DForOutWhenUnconnected=off
  wires:
  Service_Vehicle_Illumination[]/1 -> Mux/8
  Emergency_Vehicle_Illumination[]/1 -> Mux/7
  License_Plate_Illumination_Rear[]/1 -> Mux/5
  Front_Fog_Light[]/1 -> Mux/3
  Rear_Fog_Light[]/1 -> Mux/6
  Brake[]/1 -> Mux/10
  Head_Light[]/1 -> Mux/4
  High_Beam[]/1 -> Mux/1
  Reversing_Light[]/1 -> Mux/2
  Indicator_State[]/1(Indicator_State[]) -> Mux/9
  Mux/1 -> Lightstates[]/1  "LightStates[]"
  Fellow_Indicator_State[]/1 -> Indicator_State[]/1(Fellow_TurnLights[])

== system ASM_Traffic_new/Environment/GroundTruth/UserInterface/PAR_Plant/Fellow_Vehicles/Lightstates_Fellow21 ==
  Fellow_Indicator_State[] : Inport
  Brake[] : Constant  Tag=AD:ASM_Sw_SpeedLimit_Source[1Manual|2RoadScenery]  Value=2
  Emergency_Vehicle_Illumination[] : Constant  Tag=AD:ASM_Sw_SpeedLimit_Source[1Manual|2RoadScenery]  Value=2
  Front_Fog_Light[] : Constant  Tag=AD:ASM_Sw_SpeedLimit_Source[1Manual|2RoadScenery]  Value=2
  Head_Light[] : Constant  Tag=AD:ASM_Sw_SpeedLimit_Source[1Manual|2RoadScenery]  Value=2
  High_Beam[] : Constant  Tag=AD:ASM_Sw_SpeedLimit_Source[1Manual|2RoadScenery]  Value=2
  Indicator_State[] : Subsystem
  License_Plate_Illumination_Rear[] : Constant  Tag=AD:ASM_Sw_SpeedLimit_Source[1Manual|2RoadScenery]  Value=2
  Mux : Mux  Inputs=10
  Rear_Fog_Light[] : Constant  Tag=AD:ASM_Sw_SpeedLimit_Source[1Manual|2RoadScenery]  Value=2
  Reversing_Light[] : Constant  Tag=AD:ASM_Sw_SpeedLimit_Source[1Manual|2RoadScenery]  Value=2
  Service_Vehicle_Illumination[] : Constant  Tag=AD:ASM_Sw_SpeedLimit_Source[1Manual|2RoadScenery]  Value=2
  Lightstates[] : Outport  VectorParamsAs1DForOutWhenUnconnected=off
  wires:
  Fellow_Indicator_State[]/1 -> Indicator_State[]/1(Fellow_TurnLights[])
  Mux/1 -> Lightstates[]/1  "LightStates[]"
  Indicator_State[]/1(Indicator_State[]) -> Mux/9
  Reversing_Light[]/1 -> Mux/2
  High_Beam[]/1 -> Mux/1
  Head_Light[]/1 -> Mux/4
  Brake[]/1 -> Mux/10
  Rear_Fog_Light[]/1 -> Mux/6
  Front_Fog_Light[]/1 -> Mux/3
  License_Plate_Illumination_Rear[]/1 -> Mux/5
  Emergency_Vehicle_Illumination[]/1 -> Mux/7
  Service_Vehicle_Illumination[]/1 -> Mux/8

== system ASM_Traffic_new/Environment/GroundTruth/UserInterface/PAR_Plant/Fellow_Vehicles/Lightstates_Fellow22 ==
  Fellow_Indicator_State[] : Inport
  Brake[] : Constant  Tag=AD:ASM_Sw_SpeedLimit_Source[1Manual|2RoadScenery]  Value=2
  Emergency_Vehicle_Illumination[] : Constant  Tag=AD:ASM_Sw_SpeedLimit_Source[1Manual|2RoadScenery]  Value=2
  Front_Fog_Light[] : Constant  Tag=AD:ASM_Sw_SpeedLimit_Source[1Manual|2RoadScenery]  Value=2
  Head_Light[] : Constant  Tag=AD:ASM_Sw_SpeedLimit_Source[1Manual|2RoadScenery]  Value=2
  High_Beam[] : Constant  Tag=AD:ASM_Sw_SpeedLimit_Source[1Manual|2RoadScenery]  Value=2
  Indicator_State[] : Subsystem
  License_Plate_Illumination_Rear[] : Constant  Tag=AD:ASM_Sw_SpeedLimit_Source[1Manual|2RoadScenery]  Value=2
  Mux : Mux  Inputs=10
  Rear_Fog_Light[] : Constant  Tag=AD:ASM_Sw_SpeedLimit_Source[1Manual|2RoadScenery]  Value=2
  Reversing_Light[] : Constant  Tag=AD:ASM_Sw_SpeedLimit_Source[1Manual|2RoadScenery]  Value=2
  Service_Vehicle_Illumination[] : Constant  Tag=AD:ASM_Sw_SpeedLimit_Source[1Manual|2RoadScenery]  Value=2
  Lightstates[] : Outport  VectorParamsAs1DForOutWhenUnconnected=off
  wires:
  Service_Vehicle_Illumination[]/1 -> Mux/8
  Emergency_Vehicle_Illumination[]/1 -> Mux/7
  License_Plate_Illumination_Rear[]/1 -> Mux/5
  Front_Fog_Light[]/1 -> Mux/3
  Rear_Fog_Light[]/1 -> Mux/6
  Brake[]/1 -> Mux/10
  Head_Light[]/1 -> Mux/4
  High_Beam[]/1 -> Mux/1
  Reversing_Light[]/1 -> Mux/2
  Indicator_State[]/1(Indicator_State[]) -> Mux/9
  Mux/1 -> Lightstates[]/1  "LightStates[]"
  Fellow_Indicator_State[]/1 -> Indicator_State[]/1(Fellow_TurnLights[])

== system ASM_Traffic_new/Environment/GroundTruth/UserInterface/PAR_Plant/Fellow_Vehicles/Lightstates_Fellow23 ==
  Fellow_Indicator_State[] : Inport
  Brake[] : Constant  Tag=AD:ASM_Sw_SpeedLimit_Source[1Manual|2RoadScenery]  Value=2
  Emergency_Vehicle_Illumination[] : Constant  Tag=AD:ASM_Sw_SpeedLimit_Source[1Manual|2RoadScenery]  Value=2
  Front_Fog_Light[] : Constant  Tag=AD:ASM_Sw_SpeedLimit_Source[1Manual|2RoadScenery]  Value=2
  Head_Light[] : Constant  Tag=AD:ASM_Sw_SpeedLimit_Source[1Manual|2RoadScenery]  Value=2
  High_Beam[] : Constant  Tag=AD:ASM_Sw_SpeedLimit_Source[1Manual|2RoadScenery]  Value=2
  Indicator_State[] : Subsystem
  License_Plate_Illumination_Rear[] : Constant  Tag=AD:ASM_Sw_SpeedLimit_Source[1Manual|2RoadScenery]  Value=2
  Mux : Mux  Inputs=10
  Rear_Fog_Light[] : Constant  Tag=AD:ASM_Sw_SpeedLimit_Source[1Manual|2RoadScenery]  Value=2
  Reversing_Light[] : Constant  Tag=AD:ASM_Sw_SpeedLimit_Source[1Manual|2RoadScenery]  Value=2
  Service_Vehicle_Illumination[] : Constant  Tag=AD:ASM_Sw_SpeedLimit_Source[1Manual|2RoadScenery]  Value=2
  Lightstates[] : Outport  VectorParamsAs1DForOutWhenUnconnected=off
  wires:
  Fellow_Indicator_State[]/1 -> Indicator_State[]/1(Fellow_TurnLights[])
  Mux/1 -> Lightstates[]/1  "LightStates[]"
  Indicator_State[]/1(Indicator_State[]) -> Mux/9
  Reversing_Light[]/1 -> Mux/2
  High_Beam[]/1 -> Mux/1
  Head_Light[]/1 -> Mux/4
  Brake[]/1 -> Mux/10
  Rear_Fog_Light[]/1 -> Mux/6
  Front_Fog_Light[]/1 -> Mux/3
  License_Plate_Illumination_Rear[]/1 -> Mux/5
  Emergency_Vehicle_Illumination[]/1 -> Mux/7
  Service_Vehicle_Illumination[]/1 -> Mux/8

== system ASM_Traffic_new/Environment/GroundTruth/UserInterface/PAR_Plant/Fellow_Vehicles/Lightstates_Fellow24 ==
  Fellow_Indicator_State[] : Inport
  Brake[] : Constant  Tag=AD:ASM_Sw_SpeedLimit_Source[1Manual|2RoadScenery]  Value=2
  Emergency_Vehicle_Illumination[] : Constant  Tag=AD:ASM_Sw_SpeedLimit_Source[1Manual|2RoadScenery]  Value=2
  Front_Fog_Light[] : Constant  Tag=AD:ASM_Sw_SpeedLimit_Source[1Manual|2RoadScenery]  Value=2
  Head_Light[] : Constant  Tag=AD:ASM_Sw_SpeedLimit_Source[1Manual|2RoadScenery]  Value=2
  High_Beam[] : Constant  Tag=AD:ASM_Sw_SpeedLimit_Source[1Manual|2RoadScenery]  Value=2
  Indicator_State[] : Subsystem
  License_Plate_Illumination_Rear[] : Constant  Tag=AD:ASM_Sw_SpeedLimit_Source[1Manual|2RoadScenery]  Value=2
  Mux : Mux  Inputs=10
  Rear_Fog_Light[] : Constant  Tag=AD:ASM_Sw_SpeedLimit_Source[1Manual|2RoadScenery]  Value=2
  Reversing_Light[] : Constant  Tag=AD:ASM_Sw_SpeedLimit_Source[1Manual|2RoadScenery]  Value=2
  Service_Vehicle_Illumination[] : Constant  Tag=AD:ASM_Sw_SpeedLimit_Source[1Manual|2RoadScenery]  Value=2
  Lightstates[] : Outport  VectorParamsAs1DForOutWhenUnconnected=off
  wires:
  Service_Vehicle_Illumination[]/1 -> Mux/8
  Emergency_Vehicle_Illumination[]/1 -> Mux/7
  License_Plate_Illumination_Rear[]/1 -> Mux/5
  Front_Fog_Light[]/1 -> Mux/3
  Rear_Fog_Light[]/1 -> Mux/6
  Brake[]/1 -> Mux/10
  Head_Light[]/1 -> Mux/4
  High_Beam[]/1 -> Mux/1
  Reversing_Light[]/1 -> Mux/2
  Indicator_State[]/1(Indicator_State[]) -> Mux/9
  Mux/1 -> Lightstates[]/1  "LightStates[]"
  Fellow_Indicator_State[]/1 -> Indicator_State[]/1(Fellow_TurnLights[])

== system ASM_Traffic_new/Environment/GroundTruth/UserInterface/PAR_Plant/Fellow_Vehicles/Lightstates_Fellow25 ==
  Fellow_Indicator_State[] : Inport
  Brake[] : Constant  Tag=AD:ASM_Sw_SpeedLimit_Source[1Manual|2RoadScenery]  Value=2
  Emergency_Vehicle_Illumination[] : Constant  Tag=AD:ASM_Sw_SpeedLimit_Source[1Manual|2RoadScenery]  Value=2
  Front_Fog_Light[] : Constant  Tag=AD:ASM_Sw_SpeedLimit_Source[1Manual|2RoadScenery]  Value=2
  Head_Light[] : Constant  Tag=AD:ASM_Sw_SpeedLimit_Source[1Manual|2RoadScenery]  Value=2
  High_Beam[] : Constant  Tag=AD:ASM_Sw_SpeedLimit_Source[1Manual|2RoadScenery]  Value=2
  Indicator_State[] : Subsystem
  License_Plate_Illumination_Rear[] : Constant  Tag=AD:ASM_Sw_SpeedLimit_Source[1Manual|2RoadScenery]  Value=2
  Mux : Mux  Inputs=10
  Rear_Fog_Light[] : Constant  Tag=AD:ASM_Sw_SpeedLimit_Source[1Manual|2RoadScenery]  Value=2
  Reversing_Light[] : Constant  Tag=AD:ASM_Sw_SpeedLimit_Source[1Manual|2RoadScenery]  Value=2
  Service_Vehicle_Illumination[] : Constant  Tag=AD:ASM_Sw_SpeedLimit_Source[1Manual|2RoadScenery]  Value=2
  Lightstates[] : Outport  VectorParamsAs1DForOutWhenUnconnected=off
  wires:
  Fellow_Indicator_State[]/1 -> Indicator_State[]/1(Fellow_TurnLights[])
  Mux/1 -> Lightstates[]/1  "LightStates[]"
  Indicator_State[]/1(Indicator_State[]) -> Mux/9
  Reversing_Light[]/1 -> Mux/2
  High_Beam[]/1 -> Mux/1
  Head_Light[]/1 -> Mux/4
  Brake[]/1 -> Mux/10
  Rear_Fog_Light[]/1 -> Mux/6
  Front_Fog_Light[]/1 -> Mux/3
  License_Plate_Illumination_Rear[]/1 -> Mux/5
  Emergency_Vehicle_Illumination[]/1 -> Mux/7
  Service_Vehicle_Illumination[]/1 -> Mux/8

== system ASM_Traffic_new/Environment/GroundTruth/UserInterface/PAR_Plant/Fellow_Vehicles/Lightstates_Fellow26 ==
  Fellow_Indicator_State[] : Inport
  Brake[] : Constant  Tag=AD:ASM_Sw_SpeedLimit_Source[1Manual|2RoadScenery]  Value=2
  Emergency_Vehicle_Illumination[] : Constant  Tag=AD:ASM_Sw_SpeedLimit_Source[1Manual|2RoadScenery]  Value=2
  Front_Fog_Light[] : Constant  Tag=AD:ASM_Sw_SpeedLimit_Source[1Manual|2RoadScenery]  Value=2
  Head_Light[] : Constant  Tag=AD:ASM_Sw_SpeedLimit_Source[1Manual|2RoadScenery]  Value=2
  High_Beam[] : Constant  Tag=AD:ASM_Sw_SpeedLimit_Source[1Manual|2RoadScenery]  Value=2
  Indicator_State[] : Subsystem
  License_Plate_Illumination_Rear[] : Constant  Tag=AD:ASM_Sw_SpeedLimit_Source[1Manual|2RoadScenery]  Value=2
  Mux : Mux  Inputs=10
  Rear_Fog_Light[] : Constant  Tag=AD:ASM_Sw_SpeedLimit_Source[1Manual|2RoadScenery]  Value=2
  Reversing_Light[] : Constant  Tag=AD:ASM_Sw_SpeedLimit_Source[1Manual|2RoadScenery]  Value=2
  Service_Vehicle_Illumination[] : Constant  Tag=AD:ASM_Sw_SpeedLimit_Source[1Manual|2RoadScenery]  Value=2
  Lightstates[] : Outport  VectorParamsAs1DForOutWhenUnconnected=off
  wires:
  Service_Vehicle_Illumination[]/1 -> Mux/8
  Emergency_Vehicle_Illumination[]/1 -> Mux/7
  License_Plate_Illumination_Rear[]/1 -> Mux/5
  Front_Fog_Light[]/1 -> Mux/3
  Rear_Fog_Light[]/1 -> Mux/6
  Brake[]/1 -> Mux/10
  Head_Light[]/1 -> Mux/4
  High_Beam[]/1 -> Mux/1
  Reversing_Light[]/1 -> Mux/2
  Indicator_State[]/1(Indicator_State[]) -> Mux/9
  Mux/1 -> Lightstates[]/1  "LightStates[]"
  Fellow_Indicator_State[]/1 -> Indicator_State[]/1(Fellow_TurnLights[])

== system ASM_Traffic_new/Environment/GroundTruth/UserInterface/PAR_Plant/Fellow_Vehicles/Lightstates_Fellow27 ==
  Fellow_Indicator_State[] : Inport
  Brake[] : Constant  Tag=AD:ASM_Sw_SpeedLimit_Source[1Manual|2RoadScenery]  Value=2
  Emergency_Vehicle_Illumination[] : Constant  Tag=AD:ASM_Sw_SpeedLimit_Source[1Manual|2RoadScenery]  Value=2
  Front_Fog_Light[] : Constant  Tag=AD:ASM_Sw_SpeedLimit_Source[1Manual|2RoadScenery]  Value=2
  Head_Light[] : Constant  Tag=AD:ASM_Sw_SpeedLimit_Source[1Manual|2RoadScenery]  Value=2
  High_Beam[] : Constant  Tag=AD:ASM_Sw_SpeedLimit_Source[1Manual|2RoadScenery]  Value=2
  Indicator_State[] : Subsystem
  License_Plate_Illumination_Rear[] : Constant  Tag=AD:ASM_Sw_SpeedLimit_Source[1Manual|2RoadScenery]  Value=2
  Mux : Mux  Inputs=10
  Rear_Fog_Light[] : Constant  Tag=AD:ASM_Sw_SpeedLimit_Source[1Manual|2RoadScenery]  Value=2
  Reversing_Light[] : Constant  Tag=AD:ASM_Sw_SpeedLimit_Source[1Manual|2RoadScenery]  Value=2
  Service_Vehicle_Illumination[] : Constant  Tag=AD:ASM_Sw_SpeedLimit_Source[1Manual|2RoadScenery]  Value=2
  Lightstates[] : Outport  VectorParamsAs1DForOutWhenUnconnected=off
  wires:
  Fellow_Indicator_State[]/1 -> Indicator_State[]/1(Fellow_TurnLights[])
  Mux/1 -> Lightstates[]/1  "LightStates[]"
  Indicator_State[]/1(Indicator_State[]) -> Mux/9
  Reversing_Light[]/1 -> Mux/2
  High_Beam[]/1 -> Mux/1
  Head_Light[]/1 -> Mux/4
  Brake[]/1 -> Mux/10
  Rear_Fog_Light[]/1 -> Mux/6
  Front_Fog_Light[]/1 -> Mux/3
  License_Plate_Illumination_Rear[]/1 -> Mux/5
  Emergency_Vehicle_Illumination[]/1 -> Mux/7
  Service_Vehicle_Illumination[]/1 -> Mux/8

== system ASM_Traffic_new/Environment/GroundTruth/UserInterface/PAR_Plant/Fellow_Vehicles/Lightstates_Fellow28 ==
  Fellow_Indicator_State[] : Inport
  Brake[] : Constant  Tag=AD:ASM_Sw_SpeedLimit_Source[1Manual|2RoadScenery]  Value=2
  Emergency_Vehicle_Illumination[] : Constant  Tag=AD:ASM_Sw_SpeedLimit_Source[1Manual|2RoadScenery]  Value=2
  Front_Fog_Light[] : Constant  Tag=AD:ASM_Sw_SpeedLimit_Source[1Manual|2RoadScenery]  Value=2
  Head_Light[] : Constant  Tag=AD:ASM_Sw_SpeedLimit_Source[1Manual|2RoadScenery]  Value=2
  High_Beam[] : Constant  Tag=AD:ASM_Sw_SpeedLimit_Source[1Manual|2RoadScenery]  Value=2
  Indicator_State[] : Subsystem
  License_Plate_Illumination_Rear[] : Constant  Tag=AD:ASM_Sw_SpeedLimit_Source[1Manual|2RoadScenery]  Value=2
  Mux : Mux  Inputs=10
  Rear_Fog_Light[] : Constant  Tag=AD:ASM_Sw_SpeedLimit_Source[1Manual|2RoadScenery]  Value=2
  Reversing_Light[] : Constant  Tag=AD:ASM_Sw_SpeedLimit_Source[1Manual|2RoadScenery]  Value=2
  Service_Vehicle_Illumination[] : Constant  Tag=AD:ASM_Sw_SpeedLimit_Source[1Manual|2RoadScenery]  Value=2
  Lightstates[] : Outport  VectorParamsAs1DForOutWhenUnconnected=off
  wires:
  Service_Vehicle_Illumination[]/1 -> Mux/8
  Emergency_Vehicle_Illumination[]/1 -> Mux/7
  License_Plate_Illumination_Rear[]/1 -> Mux/5
  Front_Fog_Light[]/1 -> Mux/3
  Rear_Fog_Light[]/1 -> Mux/6
  Brake[]/1 -> Mux/10
  Head_Light[]/1 -> Mux/4
  High_Beam[]/1 -> Mux/1
  Reversing_Light[]/1 -> Mux/2
  Indicator_State[]/1(Indicator_State[]) -> Mux/9
  Mux/1 -> Lightstates[]/1  "LightStates[]"
  Fellow_Indicator_State[]/1 -> Indicator_State[]/1(Fellow_TurnLights[])

== system ASM_Traffic_new/Environment/GroundTruth/UserInterface/PAR_Plant/Fellow_Vehicles/Lightstates_Fellow29 ==
  Fellow_Indicator_State[] : Inport
  Brake[] : Constant  Tag=AD:ASM_Sw_SpeedLimit_Source[1Manual|2RoadScenery]  Value=2
  Emergency_Vehicle_Illumination[] : Constant  Tag=AD:ASM_Sw_SpeedLimit_Source[1Manual|2RoadScenery]  Value=2
  Front_Fog_Light[] : Constant  Tag=AD:ASM_Sw_SpeedLimit_Source[1Manual|2RoadScenery]  Value=2
  Head_Light[] : Constant  Tag=AD:ASM_Sw_SpeedLimit_Source[1Manual|2RoadScenery]  Value=2
  High_Beam[] : Constant  Tag=AD:ASM_Sw_SpeedLimit_Source[1Manual|2RoadScenery]  Value=2
  Indicator_State[] : Subsystem
  License_Plate_Illumination_Rear[] : Constant  Tag=AD:ASM_Sw_SpeedLimit_Source[1Manual|2RoadScenery]  Value=2
  Mux : Mux  Inputs=10
  Rear_Fog_Light[] : Constant  Tag=AD:ASM_Sw_SpeedLimit_Source[1Manual|2RoadScenery]  Value=2
  Reversing_Light[] : Constant  Tag=AD:ASM_Sw_SpeedLimit_Source[1Manual|2RoadScenery]  Value=2
  Service_Vehicle_Illumination[] : Constant  Tag=AD:ASM_Sw_SpeedLimit_Source[1Manual|2RoadScenery]  Value=2
  Lightstates[] : Outport  VectorParamsAs1DForOutWhenUnconnected=off
  wires:
  Fellow_Indicator_State[]/1 -> Indicator_State[]/1(Fellow_TurnLights[])
  Mux/1 -> Lightstates[]/1  "LightStates[]"
  Indicator_State[]/1(Indicator_State[]) -> Mux/9
  Reversing_Light[]/1 -> Mux/2
  High_Beam[]/1 -> Mux/1
  Head_Light[]/1 -> Mux/4
  Brake[]/1 -> Mux/10
  Rear_Fog_Light[]/1 -> Mux/6
  Front_Fog_Light[]/1 -> Mux/3
  License_Plate_Illumination_Rear[]/1 -> Mux/5
  Emergency_Vehicle_Illumination[]/1 -> Mux/7
  Service_Vehicle_Illumination[]/1 -> Mux/8

== system ASM_Traffic_new/Environment/GroundTruth/UserInterface/PAR_Plant/Fellow_Vehicles/Lightstates_Fellow3 ==
  Fellow_Indicator_State[] : Inport
  Brake[] : Constant  Tag=AD:ASM_Sw_SpeedLimit_Source[1Manual|2RoadScenery]  Value=2
  Emergency_Vehicle_Illumination[] : Constant  Tag=AD:ASM_Sw_SpeedLimit_Source[1Manual|2RoadScenery]  Value=2
  Front_Fog_Light[] : Constant  Tag=AD:ASM_Sw_SpeedLimit_Source[1Manual|2RoadScenery]  Value=2
  Head_Light[] : Constant  Tag=AD:ASM_Sw_SpeedLimit_Source[1Manual|2RoadScenery]  Value=2
  High_Beam[] : Constant  Tag=AD:ASM_Sw_SpeedLimit_Source[1Manual|2RoadScenery]  Value=2
  Indicator_State[] : Subsystem
  License_Plate_Illumination_Rear[] : Constant  Tag=AD:ASM_Sw_SpeedLimit_Source[1Manual|2RoadScenery]  Value=2
  Mux : Mux  Inputs=10
  Rear_Fog_Light[] : Constant  Tag=AD:ASM_Sw_SpeedLimit_Source[1Manual|2RoadScenery]  Value=2
  Reversing_Light[] : Constant  Tag=AD:ASM_Sw_SpeedLimit_Source[1Manual|2RoadScenery]  Value=2
  Service_Vehicle_Illumination[] : Constant  Tag=AD:ASM_Sw_SpeedLimit_Source[1Manual|2RoadScenery]  Value=2
  Lightstates[] : Outport  VectorParamsAs1DForOutWhenUnconnected=off
  wires:
  Fellow_Indicator_State[]/1 -> Indicator_State[]/1(Fellow_TurnLights[])
  Mux/1 -> Lightstates[]/1  "LightStates[]"
  Indicator_State[]/1(Indicator_State[]) -> Mux/9
  Reversing_Light[]/1 -> Mux/2
  High_Beam[]/1 -> Mux/1
  Head_Light[]/1 -> Mux/4
  Brake[]/1 -> Mux/10
  Rear_Fog_Light[]/1 -> Mux/6
  Front_Fog_Light[]/1 -> Mux/3
  License_Plate_Illumination_Rear[]/1 -> Mux/5
  Emergency_Vehicle_Illumination[]/1 -> Mux/7
  Service_Vehicle_Illumination[]/1 -> Mux/8
